simulink model "mcb_ipmsm_fwc_qep_f28379d"  (R2024b)
settings: Solver=FixedStepDiscrete  StartTime=0.0  StopTime=3  RelTol=1e-3  EnableMultiTasking=on
InitFcn:
  | mcb_ipmsm_fwc_qep_f28379d_data;
model workspace (MAT data in the model file):
  encoderResolution = 2000
  hallOffset = '0.5'
  indexOffset = 850
  polePairs = '4'
values from neighbouring files (symbols this model uses):
  dataType = 'single'    [mcb_e11_nonlin_fwc_data.m]    (also in mcb_e11_nonlin_setup.m; mcb_e11_params.m; mcb_ipmsm_fwc_qep_f28379d_data.m)
  inverter =     [e11_pmsmlut_full.mat]    (also in mcb_e11_nonlin_fwc_data.m = mcb_SetInverterParameters('BoostXL-DRV8305'); mcb_e11_nonlin_setup.m = S.inverter; mcb_ipmsm_fwc_qep_f28379d_data.m = mcb_SetInverterParameters('BoostXL-DRV8305'))
  lambda_pm = 0.0758825560532    [e11_pmsm_lut_data.mat]
  maxMotorCurrent = pmsm.I_rated    [mcb_e11_nonlin_fwc_data.m]    (also in mcb_e11_nonlin_setup.m; mcb_ipmsm_fwc_qep_f28379d_data.m)
  PI_params = mcb_SetControllerParameters(pmsm, inverter, PU_System, T_pwm, Ts, Ts_speed, Delays)    [mcb_e11_nonlin_fwc_data.m]    (also in mcb_e11_nonlin_setup.m; mcb_ipmsm_fwc_qep_f28379d_data.m = mcb_SetControllerParameters(pmsm,inverter,PU_System,T_pwm,Ts)
  pmsm = struct('I_rated', 433)    [e11_build_pmsmlut.m]    (also in e11_pmsmlut_full.mat = ; mcb_e11_nonlin_fwc_data.m = mcbPMSMUpdateLdLqFluxPM(pmsm, PMSMLUT, round(tmpmat(1,1)), r; mcb_e11_nonlin_setup.m = S.pmsm; mcb_ipmsm_fwc_qep_f28379d_data.m = mcb_SetPMSMMotorParameters('e11'))
  PU_System = mcb_SetPUSystem(pmsm, inverter)    [mcb_e11_nonlin_fwc_data.m]    (also in mcb_e11_nonlin_setup.m = struct(); mcb_ipmsm_fwc_qep_f28379d_data.m = mcb_SetPUSystem(pmsm,inverter))
  target = mcb_SetProcessorDetails('F28379D',PWM_frequency)    [mcb_ipmsm_fwc_qep_f28379d_data.m]
  Ts = T_pwm    (= 5e-05)    [mcb_e11_nonlin_fwc_data.m]    (also in mcb_e11_nonlin_setup.m; mcb_e11_params.m = ELEC.T_pwm; mcb_ipmsm_fwc_qep_f28379d_data.m)
  Ts_motor = T_pwm/2    (= 2.5e-05)    [mcb_e11_nonlin_fwc_data.m]    (also in mcb_e11_nonlin_setup.m; mcb_e11_params.m = ELEC.T_pwm/2; mcb_ipmsm_fwc_qep_f28379d_data.m)
  Ts_simulink = T_pwm/2    (= 2.5e-05)    [mcb_e11_nonlin_fwc_data.m]    (also in mcb_e11_nonlin_setup.m; mcb_e11_params.m = ELEC.T_pwm/2; mcb_ipmsm_fwc_qep_f28379d_data.m)
  Ts_speed = 30*Ts    (= 0.0015)    [mcb_e11_nonlin_fwc_data.m]    (also in mcb_e11_nonlin_setup.m; mcb_e11_params.m = 30*Ts; mcb_ipmsm_fwc_qep_f28379d_data.m)
undefined symbols (not defined in the file or in its folder): Down, GPTRIP1SEL, GPTRIP2SEL, TZ1, TZ2, Up
libraries: mcbcontrolslib x13, simulink x11, c280xlib x8, c2802xlib x7, slpidlib x4, mcbpositiondecoderlib x3, c2837xDlib x3, mcbpmsmnonlinearlib x2, svdschedulerlib x2, svdutilitieslib x1, mcbplantlib x1, autolibpmsminterior x1
(part 3 of 3)

== system mcb_ipmsm_fwc_qep_f28379d/Hardware Init/Variant Subsystem/Code Generation/Calculate ADC Offset  ==
  Enable : EnablePort
  Constant : Constant  Value=8
  Constant1 : Constant  Value=inverter.CtSensOffsetMax  OutDataTypeStr=Inherit: Inherit via back propagation
  Constant2 : Constant  Value=inverter.CtSensOffsetMin  OutDataTypeStr=Inherit: Inherit via back propagation
  Divide : Product  Inputs=*/  OutDataTypeStr=uint16
  Divide1 : Product  Inputs=*/  OutDataTypeStr=uint16
  For Iterator Subsystem : Subsystem  TreatAsAtomicUnit=on
  If : If  NumInputs=3  IfExpression=u1 > u3 & u1 < u2
  If Action Subsystem : Subsystem  TreatAsAtomicUnit=on
  If Action Subsystem1 : Subsystem  TreatAsAtomicUnit=on
  If Action Subsystem2 : Subsystem  TreatAsAtomicUnit=on
  If Action Subsystem3 : Subsystem  TreatAsAtomicUnit=on
  If1 : If  NumInputs=3  IfExpression=u1 > u3 & u1 < u2
  wires:
  For Iterator Subsystem/2(Out2) -> Divide1/1
  Divide/1 -> If Action Subsystem/1(In1), If/1
  For Iterator Subsystem/1(Out1) -> Divide/1
  Constant/1 -> Divide/2, Divide1/2
  Divide1/1 -> If1/1, If Action Subsystem2/1(In1)
  If/1 -> If Action Subsystem/Action
  If/2 -> If Action Subsystem1/Action
  If1/1 -> If Action Subsystem2/Action
  If1/2 -> If Action Subsystem3/Action
  Constant1/1 -> If1/2, If/2
  Constant2/1 -> If/3, If1/3

== system mcb_ipmsm_fwc_qep_f28379d/Hardware Init/Variant Subsystem/Code Generation/DRV Enable ==
  note: Enable DRV8305 in CPU1
  In : Inport
  DRV830x Enable : Constant  OutDataTypeStr=uint16  SampleTime=-1
  Demux : Demux  Outputs=2
  Digital Output : c2837xDlib/Digital Output  Priority=10  GPIO_Number=GPIO120~GPIO127  GPIO_Bit0=off  GPIO_BIT0_Toggle=off  GPIO_Bit1=off  GPIO_BIT1_Toggle=off  GPIO_Bit2=off  GPIO_BIT2_Toggle=off  GPIO_Bit3=off  GPIO_BIT3_Toggle=off  GPIO_Bit4=on  GPIO_BIT4_Toggle=off  GPIO_Bit5=off  GPIO_BIT5_Toggle=off  GPIO_Bit6=off  GPIO_BIT6_Toggle=off  GPIO_Bit7=off  GPIO_BIT7_Toggle=off
  Display : Display
      settings: Format=hex (Stored Integer)
  Display1 : Display
      settings: Format=hex (Stored Integer)
  SPI Master Transfer : c280xlib/SPI Controller Transfer  SPISelect=SPI_A  ClockPolarity=Rising_edge  ClockPhase=No_delay  SPIModule=uint32(0)  Mode=Master  BusSpeed=uint32(1000000)  FirstBitToTransfer=Most significant bit (MSB)  ClockMode=0  BlockFunction=Transfer  EnableRegisterAddress=off  RegisterAddress=0  OutputDataType=int8  OutputDataLength=1  DataBits=16  UseCustomSSPin=Provided by the SPI peripheral  ActiveLowSSPin=Active low  Pin=61
  SPI Master Transfer1 : c280xlib/SPI Controller Transfer  SPISelect=SPI_A  ClockPolarity=Rising_edge  ClockPhase=No_delay  SPIModule=uint32(0)  Mode=Master  BusSpeed=uint32(1000000)  FirstBitToTransfer=Most significant bit (MSB)  ClockMode=0  BlockFunction=Transfer  EnableRegisterAddress=off  RegisterAddress=0  OutputDataType=int8  OutputDataLength=1  DataBits=16  UseCustomSSPin=Provided by the SPI peripheral  ActiveLowSSPin=Active low  Pin=61
  wires:
  Demux/2 -> SPI Master Transfer1/1
  SPI Master Transfer1/1 -> Display1/1
  SPI Master Transfer/1 -> Display/1
  DRV830x Enable/1 -> Digital Output/1
  Demux/1 -> SPI Master Transfer/1
  In/1 -> Demux/1

== system mcb_ipmsm_fwc_qep_f28379d/Hardware Init/Variant Subsystem/Code Generation/Default ADC Offset ==
  Enable : EnablePort
  Constant : Constant  Value=inverter.CtSensAOffset  OutDataTypeStr=Inherit: Inherit via back propagation
  Constant1 : Constant  Value=inverter.CtSensBOffset  OutDataTypeStr=Inherit: Inherit via back propagation
  Data Store Write1 : DataStoreWrite  DataStoreName=IaOffset  IndexOptions=Index vector (dialog)  Indices=1  OutputSizes=1
  Data Store Write2 : DataStoreWrite  DataStoreName=IbOffset  IndexOptions=Index vector (dialog)  Indices=1  OutputSizes=1
  wires:
  Constant/1 -> Data Store Write1/1
  Constant1/1 -> Data Store Write2/1

== system mcb_ipmsm_fwc_qep_f28379d/Inverter and PMSM/Simulation/Sensor_Measurements/Get_PU  ==
  rad : Inport
  Constant2 : Constant  Value=2*pi  OutDataTypeStr=single  SampleTime=-1
  Get_PU : Gain  Gain=1/(2*pi)  RndMeth=Simplest  OutDataTypeStr=Inherit: Same as input
  Mod : Math  Operator=mod
  PU : Outport  VectorParamsAs1DForOutWhenUnconnected=off
  wires:
  rad/1 -> Mod/1
  Constant2/1 -> Mod/2
  Mod/1 -> Get_PU/1
  Get_PU/1 -> PU/1

== system mcb_ipmsm_fwc_qep_f28379d/Inverter and PMSM/Simulation/Sensor_Measurements/Wrap ==
  in : Inport
  Constant2 : Constant  OutDataTypeStr=single  SampleTime=-1
  Mod : Math  Operator=mod
  out : Outport  VectorParamsAs1DForOutWhenUnconnected=off
  wires:
  in/1 -> Mod/1
  Constant2/1 -> Mod/2
  Mod/1 -> out/1

== system mcb_ipmsm_fwc_qep_f28379d/Serial Receive/SCI_Rx/Code Generation/Data_Type_Fixed_Point ==
  SCI Receive : c280xlib/SCI Receive  sciModule=A  dataHead=''  headerCheckMaxCount=16  dataTail=''  dataType=uint32  dataLenOptions=Length via dialog  dataDim=2  maxDataLength=1  initValue=0  errOption=Output the last received value  errValue=0  sampleTime=-1  blockingMode=on  timeOut=0.00875  outputStatus=off
  Out1 : Outport
  wires:
  SCI Receive/1 -> Out1/1

== system mcb_ipmsm_fwc_qep_f28379d/Serial Receive/SCI_Rx/Code Generation/Data_Type_Float ==
  SCI Receive : c280xlib/SCI Receive  sciModule=A  dataHead=''  headerCheckMaxCount=16  dataTail=''  dataType=single  dataLenOptions=Length via dialog  dataDim=2  maxDataLength=1  initValue=0  errOption=Output the last received value  errValue=0  sampleTime=-1  blockingMode=on  timeOut=0.00875  outputStatus=off
  Out1 : Outport
  wires:
  SCI Receive/1 -> Out1/1

== system mcb_ipmsm_fwc_qep_f28379d/Serial Receive/SCI_Rx/Simulation/Data_Conditioning_Tx ==
  In1 : Inport
  In2 : Inport  Port=2
  Data_Type_Fixed_Point : Subsystem  VariantControl=~isequal(dataType, 'single')
  Data_Type_Float : Subsystem  VariantControl=isequal(dataType, 'single')
  Data : Outport

== system mcb_ipmsm_fwc_qep_f28379d/Serial Receive/SCI_Rx/Simulation/Parse ==
  Enable_PWM : Inport
  Enable_FWC : Inport  Port=2
  Debug_signals : Inport  Port=3
  Bitwise Operator : simulink/Logic and Bit Operations/Bitwise Operator  logicop=AND  UseBitMask=on  BitMask=hex2dec('0001')  BitMaskRealWorld=Stored Integer
  Bitwise Operator1 : simulink/Logic and Bit Operations/Bitwise Operator  logicop=AND  UseBitMask=on  BitMask=hex2dec('00F0')  BitMaskRealWorld=Stored Integer
  Bitwise Operator2 : simulink/Logic and Bit Operations/Bitwise Operator  logicop=AND  UseBitMask=on  BitMask=hex2dec('0002')  BitMaskRealWorld=Stored Integer
  Shift Arithmetic : ArithShift  BitShiftNumber=-1
  Shift Arithmetic1 : ArithShift  BitShiftNumber=-4
  Sum : Sum  Inputs=|+++
  Data : Outport
  wires:
  Bitwise Operator/1 -> Sum/1
  Debug_signals/1 -> Shift Arithmetic1/1
  Sum/1 -> Data/1
  Shift Arithmetic1/1 -> Bitwise Operator1/1
  Enable_PWM/1 -> Bitwise Operator/1
  Shift Arithmetic/1 -> Bitwise Operator2/1
  Bitwise Operator1/1 -> Sum/3
  Enable_FWC/1 -> Shift Arithmetic/1
  Bitwise Operator2/1 -> Sum/2

== system mcb_ipmsm_fwc_qep_f28379d/Current Control/Input Scaling/Calculate Phase Currents/Data_Type/Data_Type_Fixed_Point ==
  In1 : Inport
  Data Type Conversion : DataTypeConversion  OutDataTypeStr=fixdt(1,32,17)  ConvertRealWorld=Stored Integer (SI)  RndMeth=Simplest  SaturateOnIntegerOverflow=off
  Data Type Conversion1 : DataTypeConversion  OutDataTypeStr=dataType  RndMeth=Simplest  SaturateOnIntegerOverflow=off
  Q17 per unit conversion : ArithShift  BitShiftNumber=-6
  Out1 : Outport
  wires:
  In1/1 -> Q17 per unit conversion/1
  Data Type Conversion1/1 -> Out1/1
  Data Type Conversion/1 -> Data Type Conversion1/1
  Q17 per unit conversion/1 -> Data Type Conversion/1

== system mcb_ipmsm_fwc_qep_f28379d/Current Control/Input Scaling/Calculate Phase Currents/Data_Type/Data_Type_Float ==
  In1 : Inport
  Get ADC Voltage : Gain  Gain=target.ADC_Vref /target.ADC_MaxCount  OutDataTypeStr=dataType  RndMeth=Simplest
  Get Currents : Gain  Gain=1/inverter.ISenseVoltPerAmp  RndMeth=Simplest  OutDataTypeStr=Inherit: Same as input
  PU_Conversion : Gain  Gain=1/PU_System.I_base  RndMeth=Simplest  OutDataTypeStr=Inherit: Same as input
  Out1 : Outport
  wires:
  PU_Conversion/1 -> Out1/1
  Get Currents/1 -> PU_Conversion/1
  Get ADC Voltage/1 -> Get Currents/1
  In1/1 -> Get ADC Voltage/1

== system mcb_ipmsm_fwc_qep_f28379d/Current Control/SCI_Tx/Code Generation/Data_Conditioning_Tx/Data_Type_Fixed_Point ==
  In1 : Inport
  Data Type Conversion : DataTypeConversion  OutDataTypeStr=fixdt(1,32,28)  RndMeth=Simplest  SaturateOnIntegerOverflow=off
  Data Type Conversion3 : DataTypeConversion  OutDataTypeStr=uint32  ConvertRealWorld=Stored Integer (SI)  RndMeth=Simplest  SaturateOnIntegerOverflow=off
  Data_Log : Outport
  wires:
  In1/1 -> Data Type Conversion/1
  Data Type Conversion3/1 -> Data_Log/1
  Data Type Conversion/1 -> Data Type Conversion3/1

== system mcb_ipmsm_fwc_qep_f28379d/Current Control/SCI_Tx/Code Generation/Data_Conditioning_Tx/Data_Type_Float ==
  In1 : Inport
  Byte Pack : svdutilitieslib/Byte Pack  maskPackedDataType=uint32  datatypes={'single'}  byteAlign=4  blockPlatform=tic2000
  Data_Log : Outport
  wires:
  Byte Pack/1 -> Data_Log/1
  In1/1 -> Byte Pack/1

== system mcb_ipmsm_fwc_qep_f28379d/Current Control/SCI_Tx/Code Generation/Data_Logging/Data ==
  Data : Inport
  Data_width : Inport  Port=2
  Action Port : ActionPort
  Dummy : Constant  Value=hex2dec('0000')  OutDataTypeStr=uint32
  Mux : Mux  Inputs=2
  Data_out : Outport  VectorParamsAs1DForOutWhenUnconnected=off
  Iteration : Outport  Port=2  VectorParamsAs1DForOutWhenUnconnected=off
  wires:
  Data_width/1 -> Iteration/1
  Data/1 -> Mux/1
  Dummy/1 -> Mux/2
  Mux/1 -> Data_out/1

== system mcb_ipmsm_fwc_qep_f28379d/Current Control/SCI_Tx/Code Generation/Data_Logging/End ==
  Data : Inport
  Data_width : Inport  Port=2
  Action Port : ActionPort
  Bias : Bias  Bias=1  SaturateOnIntegerOverflow=off
  End : Constant  Value=hex2dec('45454545')  OutDataTypeStr=uint32
  Mux : Mux  Inputs=2
  Data_out : Outport  VectorParamsAs1DForOutWhenUnconnected=off
  Iteration : Outport  Port=2  VectorParamsAs1DForOutWhenUnconnected=off
  wires:
  Data/1 -> Mux/1
  Data_width/1 -> Bias/1
  Bias/1 -> Iteration/1
  End/1 -> Mux/2
  Mux/1 -> Data_out/1

== system mcb_ipmsm_fwc_qep_f28379d/Current Control/SCI_Tx/Code Generation/Data_Logging/Start ==
  Data : Inport
  Data_width : Inport  Port=2
  Action Port : ActionPort
  Bias : Bias  Bias=1  SaturateOnIntegerOverflow=off
  Mux : Mux  Inputs=2
  Start : Constant  Value=hex2dec('53535353')  OutDataTypeStr=uint32
  Data_out : Outport  VectorParamsAs1DForOutWhenUnconnected=off
  Iteration : Outport  Port=2  VectorParamsAs1DForOutWhenUnconnected=off
  wires:
  Data/1 -> Mux/2
  Data_width/1 -> Bias/1
  Bias/1 -> Iteration/1
  Start/1 -> Mux/1
  Mux/1 -> Data_out/1

== system mcb_ipmsm_fwc_qep_f28379d/Hardware Init/Variant Subsystem/Code Generation/Calculate ADC Offset /For Iterator Subsystem ==
  ADC_B_IN2 : c2802xlib/ADC  blkParamProc=C2000_Type4  ADCModule=B  samplingMode=Single sample mode  ADCResolution=12-bit (Single-ended input)  useSOC1=SOC2  useSOC2=SOC0_SOC1  SOCAcquisitionWindow=15  SOCTriggerSource=Software  SOCInterruptTrigger=No ADCINT  Ts=-1  dType=uint16  postInterrupt=off  interruptSel=ADCINT1  ADCINTContinuous=on  endma=off  chdma=1  conv1=ADCINA0  conv2=ADCINA0 and ADCINB0  conv1_Type4=ADCIN2  conv2_Type4=ADCIN0 and ADCIN1
  ADC_C_IN2 : c2802xlib/ADC  blkParamProc=C2000_Type4  ADCModule=C  samplingMode=Single sample mode  ADCResolution=12-bit (Single-ended input)  useSOC1=SOC2  useSOC2=SOC0_SOC1  SOCAcquisitionWindow=15  SOCTriggerSource=Software  SOCInterruptTrigger=No ADCINT  Ts=-1  dType=uint16  postInterrupt=off  interruptSel=ADCINT1  ADCINTContinuous=on  endma=off  chdma=1  conv1=ADCINA0  conv2=ADCINA0 and ADCINB0  conv1_Type4=ADCIN2  conv2_Type4=ADCIN0 and ADCIN1
  For Iterator : ForIterator  IterationLimit=16  IterationVariableDataType=uint16
  If : If  IfExpression=u1 > 8  ShowElse=off
  If Action Subsystem : Subsystem  TreatAsAtomicUnit=on
  Out1 : Outport
  Out2 : Outport  Port=2
  wires:
  For Iterator/1 -> If/1
  If Action Subsystem/1(Out1) -> Out1/1
  If Action Subsystem/2(Out2) -> Out2/1
  If/1 -> If Action Subsystem/Action
  ADC_C_IN2/1 -> If Action Subsystem/1(In1)
  ADC_B_IN2/1 -> If Action Subsystem/2(In2)

== system mcb_ipmsm_fwc_qep_f28379d/Hardware Init/Variant Subsystem/Code Generation/Calculate ADC Offset /If Action Subsystem ==
  In1 : Inport
  Action Port : ActionPort
  Data Store Write1 : DataStoreWrite  DataStoreName=IaOffset  IndexOptions=Index vector (dialog)  Indices=1  OutputSizes=1
  wires:
  In1/1 -> Data Store Write1/1

== system mcb_ipmsm_fwc_qep_f28379d/Hardware Init/Variant Subsystem/Code Generation/Calculate ADC Offset /If Action Subsystem1 ==
  Action Port : ActionPort
  Constant : Constant  Value=inverter.CtSensAOffset  OutDataTypeStr=Inherit: Inherit via back propagation
  Data Store Write1 : DataStoreWrite  DataStoreName=IaOffset  IndexOptions=Index vector (dialog)  Indices=1  OutputSizes=1
  wires:
  Constant/1 -> Data Store Write1/1

== system mcb_ipmsm_fwc_qep_f28379d/Hardware Init/Variant Subsystem/Code Generation/Calculate ADC Offset /If Action Subsystem2 ==
  In1 : Inport
  Action Port : ActionPort
  Data Store Write2 : DataStoreWrite  DataStoreName=IbOffset  IndexOptions=Index vector (dialog)  Indices=1  OutputSizes=1
  wires:
  In1/1 -> Data Store Write2/1

== system mcb_ipmsm_fwc_qep_f28379d/Hardware Init/Variant Subsystem/Code Generation/Calculate ADC Offset /If Action Subsystem3 ==
  Action Port : ActionPort
  Constant1 : Constant  Value=inverter.CtSensBOffset  OutDataTypeStr=Inherit: Inherit via back propagation
  Data Store Write2 : DataStoreWrite  DataStoreName=IbOffset  IndexOptions=Index vector (dialog)  Indices=1  OutputSizes=1
  wires:
  Constant1/1 -> Data Store Write2/1

== system mcb_ipmsm_fwc_qep_f28379d/Serial Receive/SCI_Rx/Simulation/Data_Conditioning_Tx/Data_Type_Fixed_Point ==
  In1 : Inport
  In2 : Inport  Port=2
  Data Type Conversion : DataTypeConversion  OutDataTypeStr=fixdt(1,32,28)  RndMeth=Simplest  SaturateOnIntegerOverflow=off
  Data Type Conversion1 : DataTypeConversion  OutDataTypeStr=uint32  RndMeth=Simplest  SaturateOnIntegerOverflow=off
  Data Type Conversion3 : DataTypeConversion  OutDataTypeStr=uint32  ConvertRealWorld=Stored Integer (SI)  RndMeth=Simplest  SaturateOnIntegerOverflow=off
  Mux : Mux  Inputs=2
  Data : Outport
  wires:
  In1/1 -> Data Type Conversion/1
  Data Type Conversion3/1 -> Mux/1
  Data Type Conversion/1 -> Data Type Conversion3/1
  In2/1 -> Data Type Conversion1/1
  Data Type Conversion1/1 -> Mux/2
  Mux/1 -> Data/1

== system mcb_ipmsm_fwc_qep_f28379d/Serial Receive/SCI_Rx/Simulation/Data_Conditioning_Tx/Data_Type_Float ==
  In1 : Inport
  In2 : Inport  Port=2
  Data Type Conversion2 : DataTypeConversion  OutDataTypeStr=single  RndMeth=Simplest  SaturateOnIntegerOverflow=off
  Mux : Mux  Inputs=2
  Data : Outport
  wires:
  In1/1 -> Mux/1
  Mux/1 -> Data/1
  In2/1 -> Data Type Conversion2/1
  Data Type Conversion2/1 -> Mux/2

== system mcb_ipmsm_fwc_qep_f28379d/Hardware Init/Variant Subsystem/Code Generation/Calculate ADC Offset /For Iterator Subsystem/If Action Subsystem ==
  In1 : Inport
  In2 : Inport  Port=2
  Action Port : ActionPort
  Memory : Memory  InheritSampleTime=on
  Memory1 : Memory  InheritSampleTime=on
  Sum : Sum
  Sum1 : Sum
  Out1 : Outport
  Out2 : Outport  Port=2
  wires:
  In1/1 -> Sum/1
  Sum/1 -> Out1/1, Memory/1
  In2/1 -> Sum1/1
  Memory/1 -> Sum/2
  Sum1/1 -> Out2/1, Memory1/1
  Memory1/1 -> Sum1/2
